simulink subsystem "plant"  (R2026a)
settings: Solver=VariableStepAuto
undefined symbols (not defined in the file): DiscIntNeverNeededParam, I, P, S
PreSaveFcn:
  | defaultToFileBlockNames(bdroot);
settings Model: Creator=kjhaydon  LastModifiedBy=kjhaydon

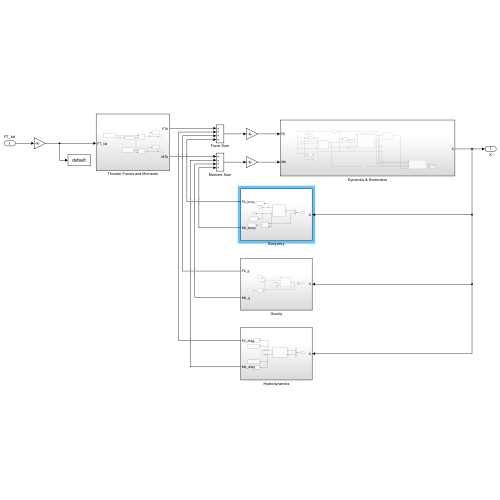
[thumbnail: Simulink's stored preview of the top-level diagram]
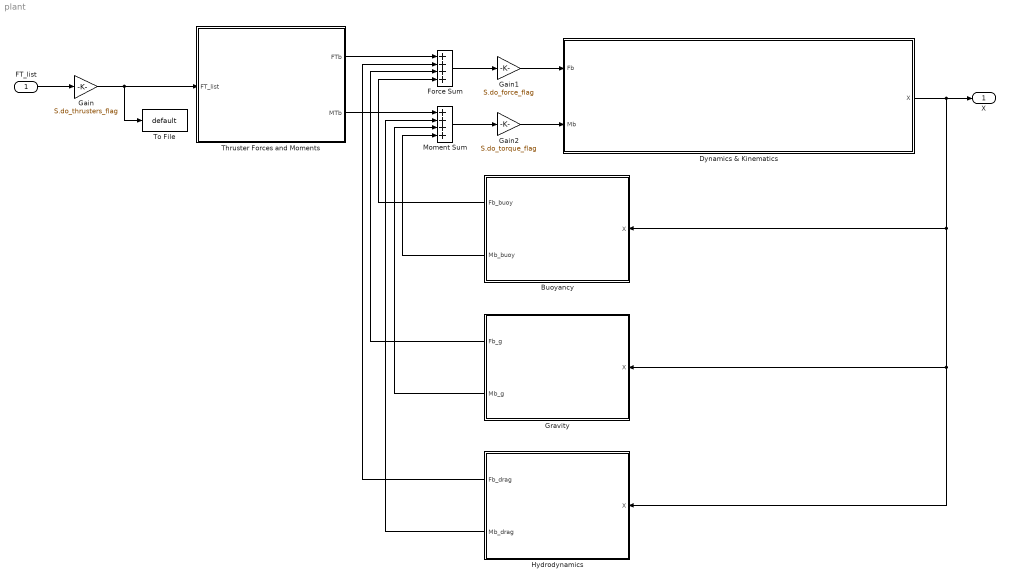
== system plant ==
  FT_list : Inport  SampleTime=S.dt_sim
  Buoyancy : Subsystem
  Dynamics & Kinematics : Subsystem
  Force Sum : Sum  Inputs=++++
  Gain : Gain  Gain=S.do_thrusters_flag
  Gain1 : Gain  Gain=S.do_force_flag
  Gain2 : Gain  Gain=S.do_torque_flag
  Gravity : Subsystem
  Hydrodynamics : Subsystem
  Moment Sum : Sum  Inputs=++++
  Thruster Forces and Moments : Subsystem
  To File : ToFile  Filename=default  MatrixName=FT_list  SaveFormat=Timeseries  SampleTime=S.dt_data
  X : Outport
  wires:
  Gravity/1(Fb_g) -> Force Sum/3
  Buoyancy/1(Fb_buoy) -> Force Sum/4
  Dynamics & Kinematics/1(X) -> Hydrodynamics/1(X), Gravity/1(X), Buoyancy/1(X), X/1
  Buoyancy/2(Mb_buoy) -> Moment Sum/4
  Gravity/2(Mb_g) -> Moment Sum/3
  Gain/1 -> Thruster Forces and Moments/1(FT_list), To File/1
  Thruster Forces and Moments/2(MTb) -> Moment Sum/1
  FT_list/1 -> Gain/1
  Thruster Forces and Moments/1(FTb) -> Force Sum/1
  Force Sum/1 -> Gain1/1
  Gain1/1 -> Dynamics & Kinematics/1(Fb)
  Moment Sum/1 -> Gain2/1
  Hydrodynamics/2(Mb_drag) -> Moment Sum/2
  Hydrodynamics/1(Fb_drag) -> Force Sum/2
  Gain2/1 -> Dynamics & Kinematics/2(Mb)

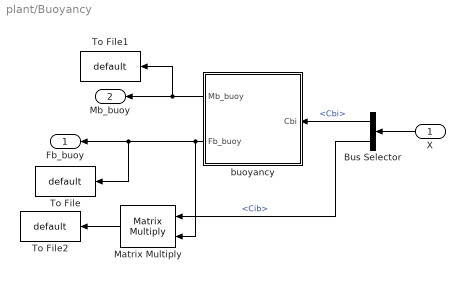
== system plant/Buoyancy ==
  X : Inport  OutDataTypeStr=Bus: X_bus
  Bus Selector : BusSelector  OutputSignals=Cbi,Cib
  Matrix Multiply : Product  Multiplication=Matrix(*)
  To File : ToFile  Filename=default  MatrixName=Fb_buoy  SaveFormat=Timeseries  SampleTime=S.dt_data
  To File1 : ToFile  Filename=default  MatrixName=Mb_buoy  SaveFormat=Timeseries  SampleTime=S.dt_data
  To File2 : ToFile  Filename=default  MatrixName=Fi_buoy  SaveFormat=Timeseries  SampleTime=S.dt_data
  buoyancy : MATLAB Function  TreatAsAtomicUnit=on
  Fb_buoy : Outport
  Mb_buoy : Outport  Port=2
  wires:
  Matrix Multiply/1 -> To File2/1
  buoyancy/1(Mb_buoy) -> To File1/1, Mb_buoy/1
  buoyancy/2(Fb_buoy) -> Matrix Multiply/2, Fb_buoy/1, To File/1
  Bus Selector/1 -> buoyancy/1(Cbi)  "<Cbi>"
  X/1 -> Bus Selector/1
  Bus Selector/2 -> Matrix Multiply/1  "<Cib>"

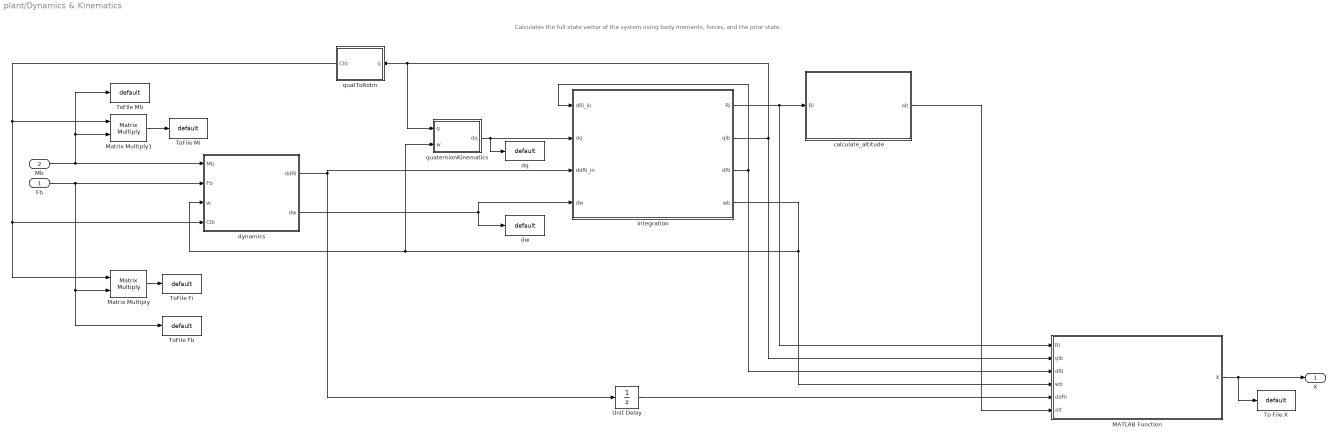
== system plant/Dynamics & Kinematics ==
  note: Calculates the full state vector of the system using body moments, forces, and the prior state.
  Fb : Inport
  Mb : Inport  Port=2
  Integration : Subsystem
  MATLAB Function : MATLAB Function  TreatAsAtomicUnit=on
  Matrix Multiply : Product  Multiplication=Matrix(*)
  Matrix Multiply1 : Product  Multiplication=Matrix(*)
  To File X : ToFile  Filename=default  MatrixName=X  SaveFormat=Timeseries  SampleTime=S.dt_data
  ToFIle Mb : ToFile  Filename=default  MatrixName=Mb  SaveFormat=Timeseries  SampleTime=S.dt_data
  ToFile Fb : ToFile  Filename=default  MatrixName=Fb  SaveFormat=Timeseries  SampleTime=S.dt_data
  ToFile Fi : ToFile  Filename=default  MatrixName=Fi  SaveFormat=Timeseries  SampleTime=S.dt_data
  ToFile Mi : ToFile  Filename=default  MatrixName=Mi  SaveFormat=Timeseries  SampleTime=S.dt_data
  Unit Delay : UnitDelay  InitialCondition=[0;0;0]  SampleTime=-1
  calculate_altitude : Subsystem
  dq : ToFile  Filename=default  MatrixName=dq  SaveFormat=Timeseries  SampleTime=S.dt_data
  dw : ToFile  Filename=default  MatrixName=dw  SaveFormat=Timeseries  SampleTime=S.dt_data
  dynamics : MATLAB Function  TreatAsAtomicUnit=on
  quatToRotm : MATLAB Function  TreatAsAtomicUnit=on
  quaternionKinematics : MATLAB Function  TreatAsAtomicUnit=on
  X : Outport  OutDataTypeStr=Bus: X_bus
  wires:
  Matrix Multiply1/1 -> ToFile Mi/1
  Unit Delay/1 -> MATLAB Function/5(ddRi)
  MATLAB Function/1(X) -> X/1, To File X/1
  Matrix Multiply/1 -> ToFile Fi/1
  quatToRotm/1(Cib) -> dynamics/4(Cib), Matrix Multiply/1, Matrix Multiply1/1
  Fb/1 -> Matrix Multiply/2, ToFile Fb/1, dynamics/2(Fb)
  dynamics/1(ddRi) -> Unit Delay/1, Integration/3(ddRi_in)
  dynamics/2(dw) -> dw/1, Integration/4(dw)
  Integration/3(dRi) -> Integration/1(dRi_in), MATLAB Function/3(dRi)
  quaternionKinematics/1(dq) -> Integration/2(dq), dq/1
  Integration/1(Ri) -> calculate_altitude/1(Ri), MATLAB Function/1(Ri)
  Mb/1 -> dynamics/1(Mb), ToFIle Mb/1, Matrix Multiply1/2
  Integration/2(qib) -> quatToRotm/1(q), quaternionKinematics/1(q), MATLAB Function/2(qib)
  Integration/4(wb) -> MATLAB Function/4(wb), dynamics/3(w), quaternionKinematics/2(w)
  calculate_altitude/1(alt) -> MATLAB Function/6(alt)

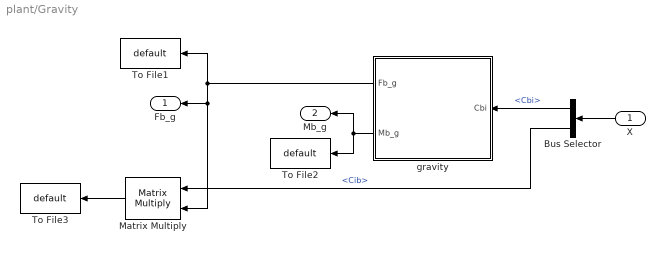
== system plant/Gravity ==
  X : Inport  OutDataTypeStr=Bus: X_bus
  Bus Selector : BusSelector  OutputSignals=Cbi,Cib
  Matrix Multiply : Product  Multiplication=Matrix(*)
  To File1 : ToFile  Filename=default  MatrixName=Fb_g  SaveFormat=Timeseries  SampleTime=S.dt_data
  To File2 : ToFile  Filename=default  MatrixName=Mb_g  SaveFormat=Timeseries  SampleTime=S.dt_data
  To File3 : ToFile  Filename=default  MatrixName=Fi_g  SaveFormat=Timeseries  SampleTime=S.dt_data
  gravity : MATLAB Function  TreatAsAtomicUnit=on
  Fb_g : Outport
  Mb_g : Outport  Port=2
  wires:
  Bus Selector/2 -> Matrix Multiply/1  "<Cib>"
  Bus Selector/1 -> gravity/1(Cbi)  "<Cbi>"
  X/1 -> Bus Selector/1
  Matrix Multiply/1 -> To File3/1
  gravity/2(Mb_g) -> Mb_g/1, To File2/1
  gravity/1(Fb_g) -> Matrix Multiply/2, Fb_g/1, To File1/1

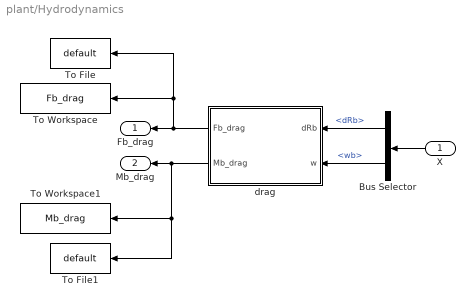
== system plant/Hydrodynamics ==
  X : Inport  OutDataTypeStr=Bus: X_bus
  Bus Selector : BusSelector  OutputSignals=dRb,wb
  To File : ToFile  Filename=default  MatrixName=Fb_drag  SaveFormat=Timeseries  SampleTime=S.dt_data
  To File1 : ToFile  Filename=default  MatrixName=Mb_drag  SaveFormat=Timeseries  SampleTime=S.dt_data
  To Workspace : ToWorkspace  VariableName=Fb_drag  SaveFormat=Timeseries  SampleTime=S.dt_data
  To Workspace1 : ToWorkspace  VariableName=Mb_drag  SaveFormat=Timeseries  SampleTime=S.dt_data
  drag : MATLAB Function  TreatAsAtomicUnit=on
  Fb_drag : Outport
  Mb_drag : Outport  Port=2
  wires:
  Bus Selector/2 -> drag/2(w)  "<wb>"
  Bus Selector/1 -> drag/1(dRb)  "<dRb>"
  X/1 -> Bus Selector/1
  drag/1(Fb_drag) -> Fb_drag/1, To File/1, To Workspace/1
  drag/2(Mb_drag) -> Mb_drag/1, To File1/1, To Workspace1/1

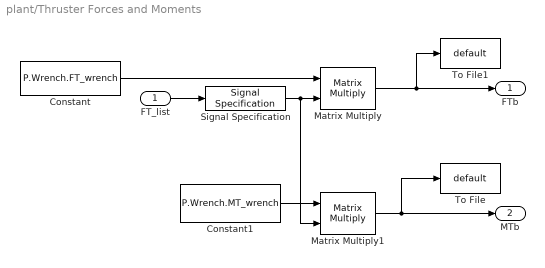
== system plant/Thruster Forces and Moments ==
  FT_list : Inport
  Constant : Constant  Value=P.Wrench.FT_wrench
  Constant1 : Constant  Value=P.Wrench.MT_wrench
  Matrix Multiply : Product  Multiplication=Matrix(*)
  Matrix Multiply1 : Product  Multiplication=Matrix(*)
  Signal Specification : SignalSpecification  Dimensions=[8 1]
  To File : ToFile  Filename=default  MatrixName=MTb  SaveFormat=Timeseries  SampleTime=S.dt_data
  To File1 : ToFile  Filename=default  MatrixName=FTb  SaveFormat=Timeseries  SampleTime=S.dt_data
  FTb : Outport
  MTb : Outport  Port=2
  wires:
  Matrix Multiply1/1 -> To File/1, MTb/1
  Matrix Multiply/1 -> To File1/1, FTb/1
  Signal Specification/1 -> Matrix Multiply1/2, Matrix Multiply/2
  FT_list/1 -> Signal Specification/1
  Constant1/1 -> Matrix Multiply1/1
  Constant/1 -> Matrix Multiply/1

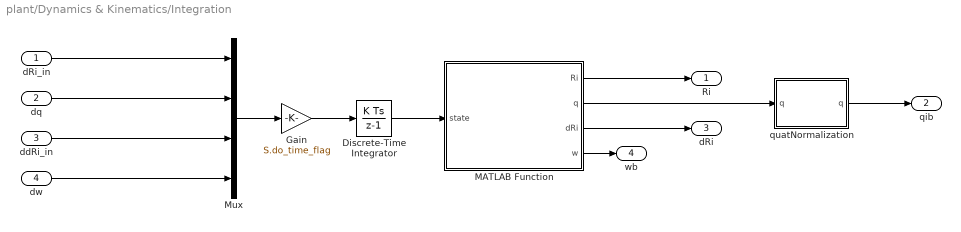
== system plant/Dynamics & Kinematics/Integration ==
  dRi_in : Inport
  dq : Inport  Port=2
  ddRi_in : Inport  Port=3
  dw : Inport  Port=4
  Discrete-Time Integrator : DiscreteIntegrator  InitialCondition=I.X0  SampleTime=-1  ICPrevOutput=DiscIntNeverNeededParam  ICPrevScaledInput=DiscIntNeverNeededParam
  Gain : Gain  Gain=S.do_time_flag
  MATLAB Function : MATLAB Function  TreatAsAtomicUnit=on
  Mux : Mux
  quatNormalization : MATLAB Function  TreatAsAtomicUnit=on
  Ri : Outport
  qib : Outport  Port=2
  dRi : Outport  Port=3
  wb : Outport  Port=4
  wires:
  Discrete-Time Integrator/1 -> MATLAB Function/1(state)
  Gain/1 -> Discrete-Time Integrator/1
  Mux/1 -> Gain/1
  MATLAB Function/2(q) -> quatNormalization/1("q ")
  quatNormalization/1(q) -> qib/1
  MATLAB Function/4(w) -> wb/1
  MATLAB Function/3(dRi) -> dRi/1
  MATLAB Function/1(Ri) -> Ri/1
  dRi_in/1 -> Mux/1
  dq/1 -> Mux/2
  dw/1 -> Mux/4
  ddRi_in/1 -> Mux/3

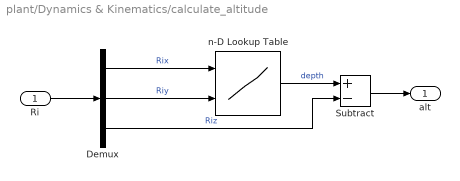
== system plant/Dynamics & Kinematics/calculate_altitude ==
  Ri : Inport
  Demux : Demux  Outputs=3
  Subtract : Sum  Inputs=+-
  n-D Lookup Table : Lookup_n-D  BreakpointsForDimension1=P.Floor.xi  BreakpointsForDimension2=P.Floor.yi  BreakpointsForDimension3=[5, 7]  Table=P.Floor.depth_surface  InternalRulePriority=Speed  RndMeth=Simplest
      settings: InputPortMap=u0,u1
  alt : Outport
  wires:
  Demux/1 -> n-D Lookup Table/1  "Rix"
  Demux/2 -> n-D Lookup Table/2  "Riy"
  n-D Lookup Table/1 -> Subtract/1  "depth"
  Subtract/1 -> alt/1
  Ri/1 -> Demux/1
  Demux/3 -> Subtract/2  "Riz"

== matlab function plant/Buoyancy/buoyancy ==
  data: Cbi input; Mb_buoy output; Fb_buoy output; P parameter; S parameter
function [Mb_buoy,Fb_buoy] = fcn(Cbi, P, S)

rho = P.Constants.rho;
V_total = P.Volume.V_total;
do_buoyancy_flag = S.do_buoyancy_flag;

R_cm2cv = P.Mass.R_o2cm - P.Volume.R_o2cv;
[Fb_buoy, Mb_buoy] =  buoyancy(Cbi, rho, V_total, R_cm2cv, do_buoyancy_flag);

== matlab function plant/Dynamics & Kinematics/Integration/MATLAB Function ==
  data: Ri output; q output; dRi output; w output; state input
function [Ri,q,dRi,w] = fcn(state)
Ri = state(1:3);
q = state(4:7);
dRi = state(8:10);
w = state(11:13);
end

== matlab function plant/Dynamics & Kinematics/Integration/quatNormalization ==
  data: q input; q output
function q = fcn(q)

q = quatNormalization(q);

== matlab function plant/Dynamics & Kinematics/MATLAB Function ==
  data: X output Bus: X_bus; Ri input; qib input; dRi input; wb input; ddRi input; alt input
function X = fcn(Ri, qib, dRi, wb, ddRi, alt)

X = packStateIntoBus(Ri, qib, dRi, wb, ddRi, alt);

== matlab function plant/Dynamics & Kinematics/dynamics ==
  data: Mb input; ddRi output; Fb input; w input; Cib input; dw output; P parameter
function [ddRi, dw] = fcn(Mb, Fb, w, Cib, P)

%unpack structure args
I = P.Mass.I;
invM = P.Mass.invM;
invI = P.Mass.invI;

[ddRi,dw] = dynamics(Mb,Fb,w,Cib,I,invM,invI);

== matlab function plant/Dynamics & Kinematics/quatToRotm ==
  data: q input; Cib output
function Cib = fcn(q)

Cib = quatToRotm(q);

== matlab function plant/Dynamics & Kinematics/quaternionKinematics ==
  data: q input; dq output; w input
function dq = fcn(q,w)

dq = quaternionKinematics(q,w);

== matlab function plant/Gravity/gravity ==
  data: Cbi input; Fb_g output; Mb_g output; P parameter; S parameter
function [Fb_g, Mb_g] = fcn(Cbi, P, S)

m = P.Mass.m;
do_gravity_flag = S.do_gravity_flag;
[Fb_g, Mb_g] = gravity(Cbi, m, do_gravity_flag);

== matlab function plant/Hydrodynamics/drag ==
  data: dRb input; Fb_drag output; w input; Mb_drag output; P parameter; S parameter
function [Fb_drag,Mb_drag] = fcn(dRb, w, P, S)

drag_wrench_lin = P.Hydro.drag_wrench_lin;
do_drag_flag = S.do_drag_flag;
drag_wrench_quad = P.Hydro.drag_wrench_quad;

[Fb_drag, Mb_drag] = drag(dRb, w, drag_wrench_lin, drag_wrench_quad, do_drag_flag);
